simulink model "MalhaAbertaSimples"  (R2025a)
settings: Solver=FixedStepDiscrete  StartTime=0.0  StopTime=0.1  FixedStep=Bancada.Ts/500  RelTol=1e-3
undefined symbols (not defined in the file or in its folder): Bancada
libraries: spsDCVoltageSourceLib x2, spsGroundLib x2, spsThreePhaseSeriesRLCBranchLib x1, spsTwoLevelConverterLib x1, spsThreePhaseVIMeasurementLib x1, spsPWMGenerator2LevelLib x1, spspowerguiLib x1, spsVoltageMeasurementLib x1
settings Model: Creator=raphateixeira  LastModifiedBy=raphateixeira
settings DataIOCC: SaveOutput=off  SignalLogging=off  SaveTime=off

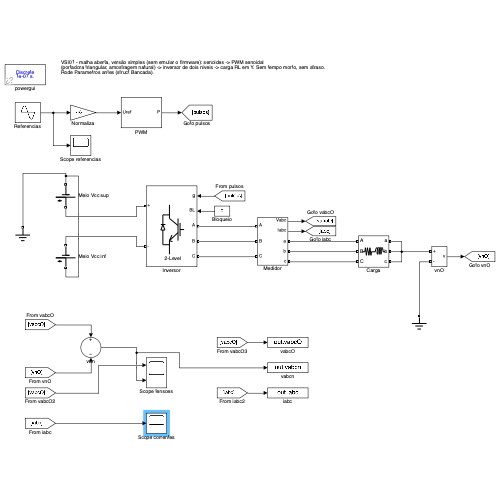
[thumbnail: Simulink's stored preview of the top-level diagram]
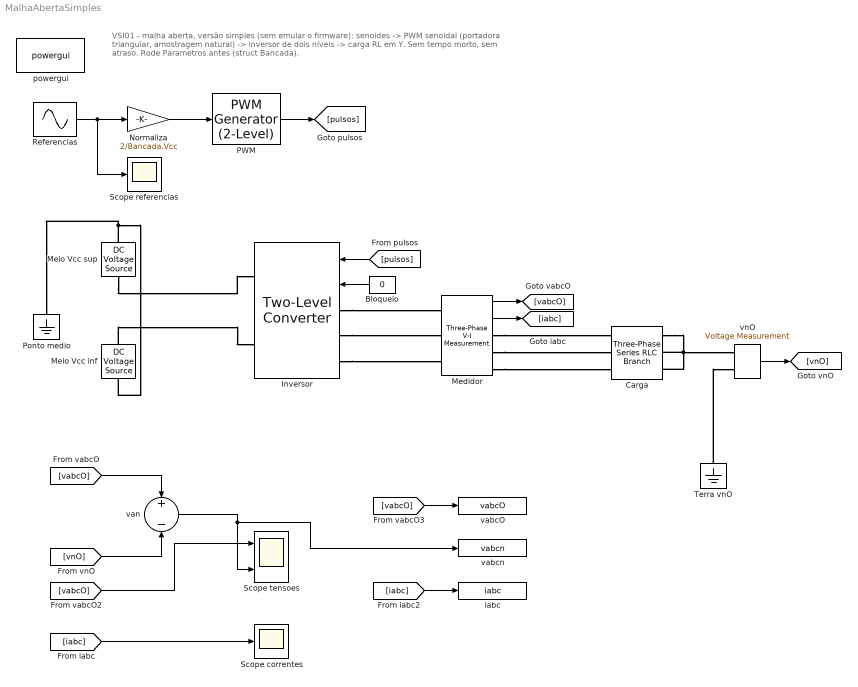
== system MalhaAbertaSimples ==
  note: VSI01 - malha aberta, versão simples (sem emular o firmware): senoides -> PWM senoidal
      | (portadora triangular, amostragem natural) -> inversor de dois níveis -> carga RL em Y. Sem tempo morto, sem atraso.
      | Rode Parametros antes (struct Bancada).
  Bloqueio : Constant  Value=0
  Carga : spsThreePhaseSeriesRLCBranchLib/Three-Phase Series RLC Branch  LConnTagsString=A|B|C  RConnTagsString=A|B|C  BranchType=RL  Resistance=Bancada.RLf + Bancada.Rc  Inductance=Bancada.Lf  Capacitance=1e-6  Measurements=None
  Inversor : spsTwoLevelConverterLib/Two-Level Converter  ModelType=Switching devices  Ron=Bancada.Ron  Rs=1e6  Cs=inf  Vforward=[0 0]  Ron_Diode=1e-3  Rs_Diode=1e6  Cs_Diode=inf  Vf_Diode=0  Rs_CurrentSource=inf  Ron_ACsource=1e-3
  Medidor : spsThreePhaseVIMeasurementLib/Three-Phase V-I Measurement  VoltageMeasurement=phase-to-ground  SetLabelV=off  LabelV=Vabc  Vpu=off  VpuLL=off  CurrentMeasurement=yes  SetLabelI=off  LabelI=Iabc  Ipu=off  Pbase=100e6  Vbase=500e3  OutputType=Complex  PhasorSimulation=off  PSBequivalent=0
  Meio Vcc inf : spsDCVoltageSourceLib/DC Voltage Source  Amplitude=Bancada.Vcc/2  Measurements=None
  Meio Vcc sup : spsDCVoltageSourceLib/DC Voltage Source  Amplitude=Bancada.Vcc/2  Measurements=None
  Normaliza : Gain  Gain=2/Bancada.Vcc
  PWM : spsPWMGenerator2LevelLib/PWM Generator (2-Level)  ModulatorType=Three-phase bridge (6 pulses)  ModulatorMode=Unsynchronized  Fc=Bancada.fPWM  Pc=0  nF=27  MinMax=[-1 1]  SamplingTechnique=Natural  ModulatingSignals=off  m=0.8  Freq=60  Phase=0  Ts=Bancada.Ts/500  ShowCarrierOutport=off
  Ponto medio : spsGroundLib/Ground  LConnTagsString=a
  Referencias : Sin  Amplitude=Bancada.Vp  Frequency=2*pi*Bancada.f  Phase=[0 -2*pi/3 2*pi/3]  SampleTime=0
  Scope correntes : Scope
      settings: ActiveDisplayYMinimum=-2.8951908092962446  ActiveDisplayYMaximum=2.8953083329956897
  Scope referencias : Scope
  Scope tensoes : Scope  NumInputPorts=2
      settings: ActiveDisplayYMinimum=-19.99993392825953  ActiveDisplayYMaximum=19.999500174784725
  Terra vnO : spsGroundLib/Ground  LConnTagsString=a
  iabc : ToWorkspace  VariableName=iabc  SaveFormat=Timeseries  SampleTime=Bancada.Tlog
  powergui : spspowerguiLib/powergui  Priority=1  SimulationMode=Discrete  SampleTime=Bancada.Ts/500  frequency=60  Iterations=50  frequencyindice=0  Pbase=100e6  ErrMax=1e-4  UnitsV=kV  UnitsW=MW  buscounter=0  FunctionMessages=off  echomessages=off  EnableUseOfTLC=off  CurrentSourceSwitches=off  DisableSnubberDevices=off  DisableRonSwitches=off  DisableVfSwitches=off  DisplayEquations=off  AutomaticDiscreteSolvers=off  SolverType=Tustin/Backward Euler (TBE)  Interpol=off  ExternalGateDelay=off  methode=off  Ts=100  x0status=blocks  SPID=on  SwTol=0  HookPort=off  NonlinearTolerance=1e-4  nMaxIteration=100  ContinueOnMaxIteration=off  RestoreLinks=warning  ResistiveCurrentMeasurement=off  Frange=[0:2:500]  Ylog=off  Xlog=on  ShowGrid=off  save=off  variable=ZData  structure=0  ZoomFFT=off  StartTime=0.0  cycles=1  DisplayStyle=1  fundamental=60  FreqAxis=off  MaxFrequency=1000  frequencyindicesteady=1  RmsSteady=1  display=off
  vabcO : ToWorkspace  VariableName=vabcO  SaveFormat=Timeseries  SampleTime=Bancada.Tlog
  vabcn : ToWorkspace  VariableName=vabcn  SaveFormat=Timeseries  SampleTime=Bancada.Tlog
  van : Sum  Inputs=+-
  vnO : spsVoltageMeasurementLib/Voltage Measurement  PhasorSimulation=off  OutputType=Complex  PSBequivalent=0
  wires:
  Referencias/1 -> Normaliza/1, Scope referencias/1
  Normaliza/1 -> PWM/1
  PWM/1 -> [pulsos]
  [pulsos] -> Inversor/1
  Bloqueio/1 -> Inversor/2
  Medidor/1 -> [vabcO]
  Medidor/2 -> [iabc]
  vnO/1 -> [vnO]
  [vabcO] -> van/1
  [vnO] -> van/2
  [vabcO] -> Scope tensoes/1
  van/1 -> Scope tensoes/2, vabcn/1
  [iabc] -> Scope correntes/1
  [vabcO] -> vabcO/1
  [iabc] -> iabc/1
  connections:
  Meio Vcc inf/RConn1 -- Meio Vcc sup/LConn1 -- Ponto medio/LConn1
  Meio Vcc sup/RConn1 -- Inversor/RConn1
  Meio Vcc inf/LConn1 -- Inversor/RConn2
  Inversor/LConn1 -- Medidor/LConn1
  Medidor/RConn1 -- Carga/LConn1
  Inversor/LConn2 -- Medidor/LConn2
  Medidor/RConn2 -- Carga/LConn2
  Inversor/LConn3 -- Medidor/LConn3
  Medidor/RConn3 -- Carga/LConn3
  Carga/RConn1 -- Carga/RConn3 -- vnO/LConn1 -- Carga/RConn2
  Terra vnO/LConn1 -- vnO/LConn2
